simulink model "XFLUID01_reference"  (R2025a)
settings: Solver=FixedStepDiscrete  StartTime=0  StopTime=16  FixedStep=0.002  RelTol=1e-3
undefined symbols (not defined in the file): bucket_reference, fluid_bulk_modulus, leak_event_time, leakage_multiplier, lift_reference, payload_mass, pump_flow_capacity, reach_reference, supply_pressure, valve_deadband
settings Model: Creator=SimuVerity Contributors  LastModifiedBy=SimuVerity Contributors

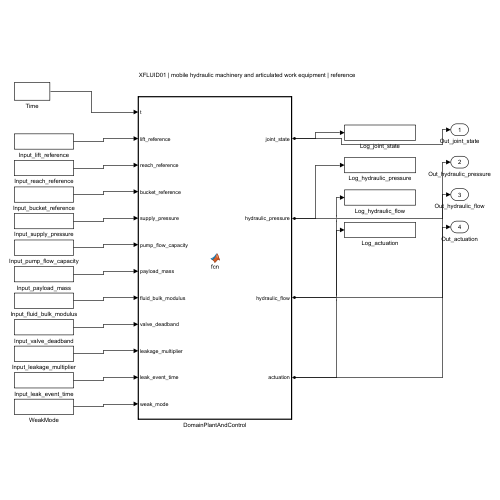
[thumbnail: Simulink's stored preview of the top-level diagram]
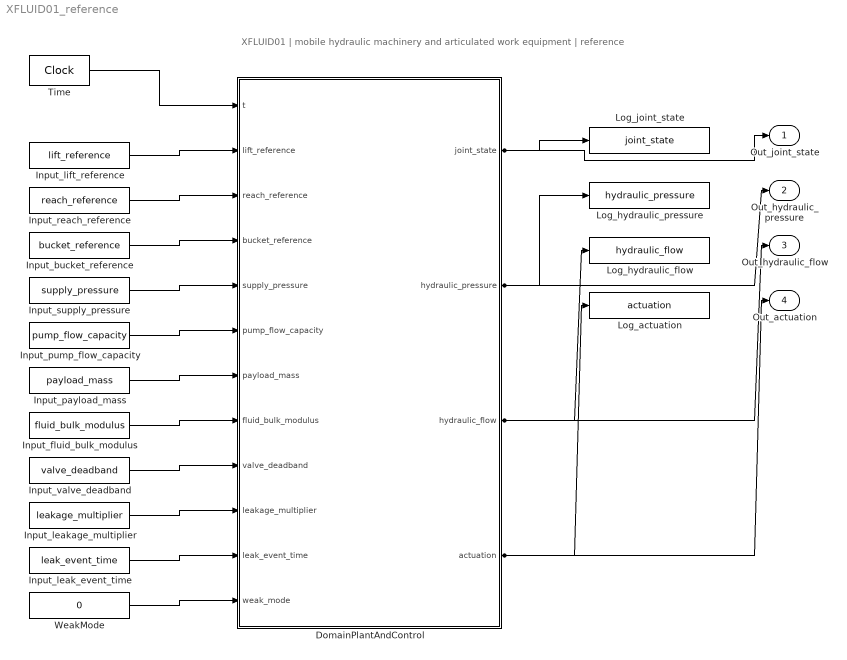
== system XFLUID01_reference ==
  note: XFLUID01 | mobile hydraulic machinery and articulated work equipment | reference
  DomainPlantAndControl : MATLAB Function  TreatAsAtomicUnit=on
  Input_bucket_reference : Constant  Value=bucket_reference
  Input_fluid_bulk_modulus : Constant  Value=fluid_bulk_modulus
  Input_leak_event_time : Constant  Value=leak_event_time
  Input_leakage_multiplier : Constant  Value=leakage_multiplier
  Input_lift_reference : Constant  Value=lift_reference
  Input_payload_mass : Constant  Value=payload_mass
  Input_pump_flow_capacity : Constant  Value=pump_flow_capacity
  Input_reach_reference : Constant  Value=reach_reference
  Input_supply_pressure : Constant  Value=supply_pressure
  Input_valve_deadband : Constant  Value=valve_deadband
  Log_actuation : ToWorkspace  VariableName=actuation  SaveFormat=Timeseries  SampleTime=-1
  Log_hydraulic_flow : ToWorkspace  VariableName=hydraulic_flow  SaveFormat=Timeseries  SampleTime=-1
  Log_hydraulic_pressure : ToWorkspace  VariableName=hydraulic_pressure  SaveFormat=Timeseries  SampleTime=-1
  Log_joint_state : ToWorkspace  VariableName=joint_state  SaveFormat=Timeseries  SampleTime=-1
  Time : DigitalClock  SampleTime=0.002
  WeakMode : Constant  Value=0
  Out_joint_state : Outport
  Out_hydraulic_pressure : Outport  Port=2
  Out_hydraulic_flow : Outport  Port=3
  Out_actuation : Outport  Port=4
  wires:
  Time/1 -> DomainPlantAndControl/1(t)
  Input_lift_reference/1 -> DomainPlantAndControl/2(lift_reference)
  Input_reach_reference/1 -> DomainPlantAndControl/3(reach_reference)
  Input_bucket_reference/1 -> DomainPlantAndControl/4(bucket_reference)
  Input_supply_pressure/1 -> DomainPlantAndControl/5(supply_pressure)
  Input_pump_flow_capacity/1 -> DomainPlantAndControl/6(pump_flow_capacity)
  Input_payload_mass/1 -> DomainPlantAndControl/7(payload_mass)
  Input_fluid_bulk_modulus/1 -> DomainPlantAndControl/8(fluid_bulk_modulus)
  Input_valve_deadband/1 -> DomainPlantAndControl/9(valve_deadband)
  Input_leakage_multiplier/1 -> DomainPlantAndControl/10(leakage_multiplier)
  Input_leak_event_time/1 -> DomainPlantAndControl/11(leak_event_time)
  WeakMode/1 -> DomainPlantAndControl/12(weak_mode)
  DomainPlantAndControl/1(joint_state) -> Log_joint_state/1, Out_joint_state/1
  DomainPlantAndControl/2(hydraulic_pressure) -> Log_hydraulic_pressure/1, Out_hydraulic_pressure/1
  DomainPlantAndControl/3(hydraulic_flow) -> Log_hydraulic_flow/1, Out_hydraulic_flow/1
  DomainPlantAndControl/4(actuation) -> Log_actuation/1, Out_actuation/1

== matlab function XFLUID01_reference/DomainPlantAndControl ==
  data: t input; joint_state output; lift_reference input; reach_reference input; bucket_reference input; supply_pressure input; pump_flow_capacity input; payload_mass input; fluid_bulk_modulus input; valve_deadband input; leakage_multiplier input; leak_event_time input; weak_mode input; hydraulic_pressure output; hydraulic_flow output; actuation output
function [joint_state,hydraulic_pressure,hydraulic_flow,actuation] = fcn(t,lift_reference,reach_reference,bucket_reference,supply_pressure,pump_flow_capacity,payload_mass,fluid_bulk_modulus,valve_deadband,leakage_multiplier,leak_event_time,weak_mode)
%#codegen
persistent q1 q2 q3 w1 w2 w3 p1 p2 p3 ps z1 z2 z3
dt=0.002; A=[0.00135,0.00120,0.00085]; lever=[0.42,0.38,0.29]; V=[0.010,0.009,0.0065];
if isempty(q1)
    q1=0; q2=0; q3=0; w1=0; w2=0; w3=0; p1=0; p2=0; p3=0;
    ps=0.92*supply_pressure; z1=0; z2=0; z3=0;
end
q=[q1,q2,q3]; w=[w1,w2,w3]; pd=[p1,p2,p3];
ref=[lift_reference,reach_reference,bucket_reference]*pi/180; e=ref-q;
event=(t>=leak_event_time && t<leak_event_time+1.2);
J=[1500+0.28*payload_mass,1250+0.42*payload_mass,430+0.11*payload_mass];
grav=[(310+payload_mass)*9.81*0.34*sin(q(1)),(250+0.72*payload_mass)*9.81*0.40*sin(q(2)),(95+0.32*payload_mass)*9.81*0.27*sin(q(3))];
coupling=260*(q(2)-q(1));
if weak_mode<0.5
    z1=min(max(z1+e(1)*dt,-1.2),1.2); z2=min(max(z2+e(2)*dt,-1.2),1.2); z3=min(max(z3+e(3)*dt,-1.2),1.2);
    tauCmd=[grav(1)-coupling,grav(2)+coupling,grav(3)]+J.*(5.0*e-4.2*w+1.8*[z1,z2,z3]);
    pDes=tauCmd./(A.*lever); pDes=min(max(pDes,-0.74*ps),0.74*ps);
    raw=2.6*(pDes-pd)/max(supply_pressure,1e6)+0.12*pDes/max(supply_pressure,1e6);
    raw=min(max(raw,-1),1);
    spool=zeros(1,3);
    for k=1:3
        if abs(raw(k))>valve_deadband,spool(k)=sign(raw(k))*(abs(raw(k))-valve_deadband)/(1-valve_deadband);end
    end
    avail=max(ps-abs(pd),2e5); qv=0.0031*spool.*sqrt(avail/18e6);
    requested=sum(abs(qv));
    if requested>pump_flow_capacity,qv=qv*(pump_flow_capacity/requested);end
    qp=A.*lever.*w;
    leakScale=[1,1+(leakage_multiplier-1)*double(event),1];
    ql=1.55e-11*pd.*leakScale+sign(pd).*max(abs(pd)-0.78*ps,0)*4.0e-10;
    dpdot=fluid_bulk_modulus./V.*(qv-qp-ql);
    pd=pd+dt*dpdot;
    tau=pd.*A.*lever;
    pumpFlow=sum(abs(qv)); util=min(pumpFlow/max(pump_flow_capacity,1e-5),1.0);
    psTarget=supply_pressure*(1-0.16*min(util,1)); ps=ps+dt*(psTarget-ps)/0.09;
    acc=[(tau(1)-780*w(1)-grav(1)+coupling)/J(1),(tau(2)-720*w(2)-grav(2)-coupling)/J(2),(tau(3)-270*w(3)-grav(3))/J(3)];
    w=w+dt*acc; q=q+dt*w;
elseif weak_mode<1.5
    % Kinematic shortcut: tracks references but has no pressure-flow-motion causality.
    acc=14*(ref-q)-6*w; w=w+dt*acc; q=q+dt*w;
    pd=0.992*pd; ps=ps+dt*(supply_pressure-ps)/0.12;
    spool=zeros(1,3);qv=zeros(1,3);qp=zeros(1,3);ql=zeros(1,3);tau=zeros(1,3);pumpFlow=0;
else
    % Developer shortcut mutant: prescribed joint motion accompanied by
    % a plausible-looking but non-causal pressure/torque ledger.
    acc=14*(ref-q)-6*w; w=w+dt*acc; q=q+dt*w;
    ps=ps+dt*(0.90*supply_pressure-ps)/0.12;
    pd=0.18*ps*[sin(0.83*t),sin(1.07*t+0.6),sin(0.71*t-0.4)];
    tau=pd.*A.*lever; spool=0.18*[sin(0.83*t),sin(1.07*t+0.6),sin(0.71*t-0.4)];
    qp=A.*lever.*w;
    leakScale=[1,1+(leakage_multiplier-1)*double(event),1];
    ql=1.55e-11*pd.*leakScale; qv=qp+ql;
    requested=sum(abs(qv));
    if requested>pump_flow_capacity,qv=qv*(pump_flow_capacity/requested);end
    pumpFlow=sum(abs(qv));
end
q1=q(1);q2=q(2);q3=q(3);w1=w(1);w2=w(2);w3=w(3);p1=pd(1);p2=pd(2);p3=pd(3);
joint_state=[q*180/pi,w*180/pi];
hydraulic_pressure=[ps,pd];
hydraulic_flow=[abs(qv),qp,ql,pumpFlow];
actuation=[spool,tau];
end
